simulink model "Sistema_Control_02"  (R2026a)
settings: Solver=VariableStepAuto
settings Model: Creator=Lorenzo  LastModifiedBy=Lorenzo

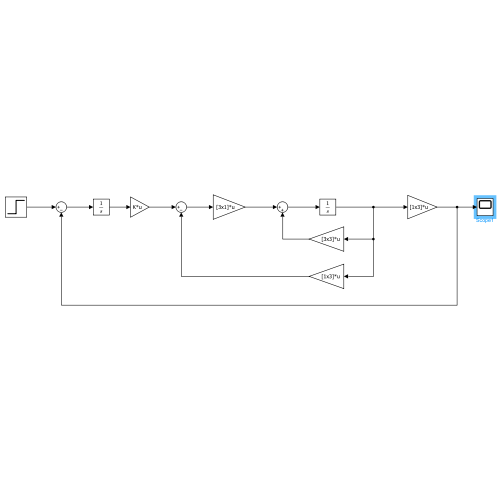
[thumbnail: Simulink's stored preview of the top-level diagram]
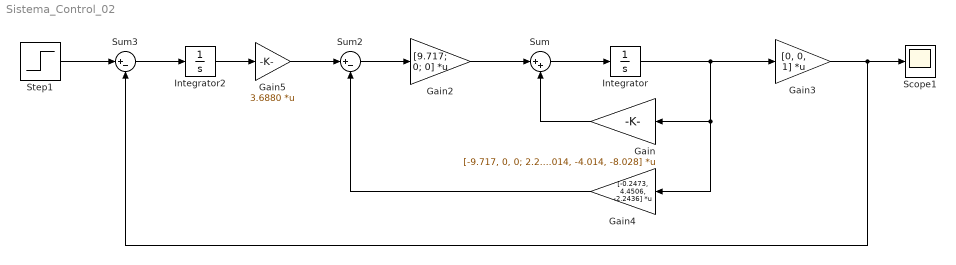
== system Sistema_Control_02 ==
  Gain : Gain  Gain=[-9.717, 0, 0; 2.209, -6.658, -2.209; 4.014, -4.014, -8.028]  Multiplication=Matrix(K*u)
  Gain2 : Gain  Gain=[9.717; 0; 0]  Multiplication=Matrix(K*u)
  Gain3 : Gain  Gain=[0, 0, 1]  Multiplication=Matrix(K*u)
  Gain4 : Gain  Gain=[-0.2473, 4.4506, -2.2436]  Multiplication=Matrix(K*u)
  Gain5 : Gain  Gain=3.6880  Multiplication=Matrix(K*u)
  Integrator : Integrator
  Integrator2 : Integrator
  Scope1 : Scope
      settings: ActiveDisplayYMinimum=-0.20111346192949198  ActiveDisplayYMaximum=1.1808392184666077
  Step1 : Step  SampleTime=0
  Sum : Sum  Inputs=|++
  Sum2 : Sum  Inputs=|+-
  Sum3 : Sum  Inputs=|+-
  wires:
  Gain2/1 -> Sum/1
  Sum/1 -> Integrator/1
  Integrator/1 -> Gain4/1, Gain/1, Gain3/1
  Gain/1 -> Sum/2
  Sum2/1 -> Gain2/1
  Gain4/1 -> Sum2/2
  Gain5/1 -> Sum2/1
  Integrator2/1 -> Gain5/1
  Step1/1 -> Sum3/1
  Sum3/1 -> Integrator2/1
  Gain3/1 -> Sum3/2, Scope1/1
